simulink model "CurrentControl"  (R2026b)
settings: Solver=VariableStepAuto
undefined symbols (not defined in the file or in its folder): currentCfg, inverterCfg
settings Model: Creator=24322  LastModifiedBy=24322

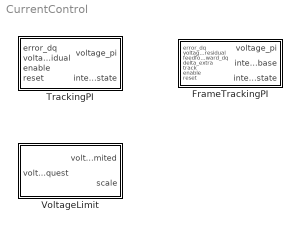
== system CurrentControl ==
  FrameTrackingPI : Subsystem  mask{currentCfg=currentCfg}
      mask prompts: currentCfg "Current controller configuration"
  TrackingPI : Subsystem
  VoltageLimit : Subsystem

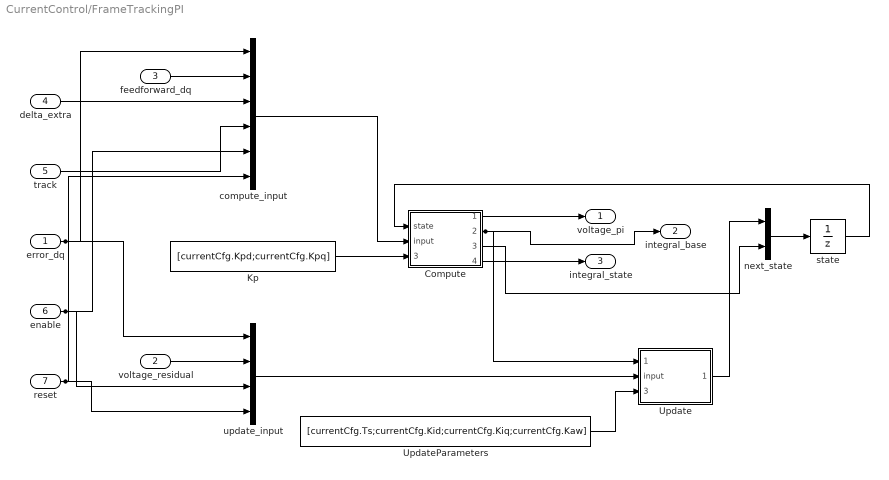
== system CurrentControl/FrameTrackingPI ==
  error_dq : Inport  SampleTime=currentCfg.Ts
  voltage_residual : Inport  Port=2  SampleTime=currentCfg.Ts
  feedforward_dq : Inport  Port=3  SampleTime=currentCfg.Ts
  delta_extra : Inport  Port=4  SampleTime=currentCfg.Ts
  track : Inport  Port=5  SampleTime=currentCfg.Ts
  enable : Inport  Port=6  SampleTime=currentCfg.Ts
  reset : Inport  Port=7  SampleTime=currentCfg.Ts
  Compute : MATLAB Function  TreatAsAtomicUnit=on
  Kp : Constant  Value=[currentCfg.Kpd;currentCfg.Kpq]
  Update : MATLAB Function  TreatAsAtomicUnit=on
  UpdateParameters : Constant  Value=[currentCfg.Ts;currentCfg.Kid;currentCfg.Kiq;currentCfg.Kaw]
  compute_input : Mux  Inputs=6
  next_state : Mux  Inputs=2
  state : UnitDelay  InitialCondition=zeros(8,1)  SampleTime=currentCfg.Ts
  update_input : Mux
  voltage_pi : Outport
  integral_base : Outport  Port=2
  integral_state : Outport  Port=3
  wires:
  voltage_residual/1 -> update_input/2
  reset/1 -> update_input/4, compute_input/6
  enable/1 -> compute_input/5, update_input/3
  track/1 -> compute_input/4
  delta_extra/1 -> compute_input/3
  feedforward_dq/1 -> compute_input/2
  error_dq/1 -> compute_input/1, update_input/1
  Compute/4(integralState) -> integral_state/1
  Compute/1(voltage) -> voltage_pi/1
  next_state/1 -> state/1
  Compute/3(history) -> next_state/2
  Update/1(nextIntegral) -> next_state/1
  UpdateParameters/1 -> Update/3(parameter)
  update_input/1 -> Update/2(input)
  Compute/2(integralBase) -> Update/1(integralBase), integral_base/1
  Kp/1 -> Compute/3(parameter)
  compute_input/1 -> Compute/2(input)
  state/1 -> Compute/1(state)

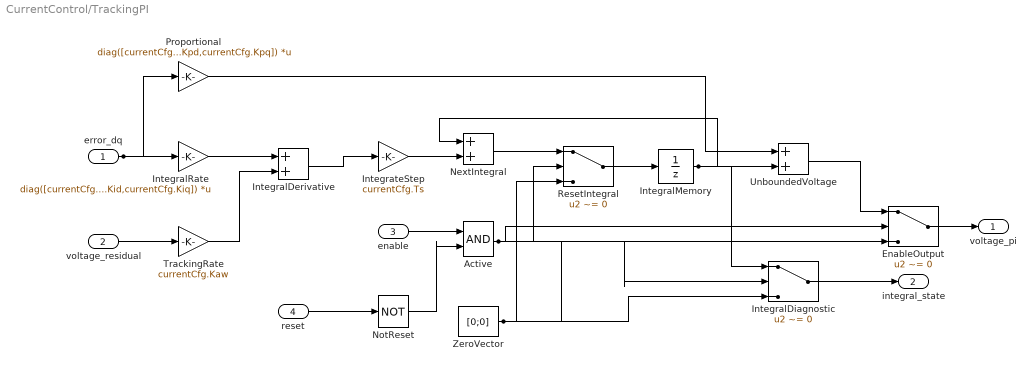
== system CurrentControl/TrackingPI ==
  error_dq : Inport
  voltage_residual : Inport  Port=2
  enable : Inport  Port=3
  reset : Inport  Port=4
  Active : Logic  IconShape=distinctive  AllPortsSameDT=off  OutDataTypeStr=boolean
  EnableOutput : Switch  Criteria=u2 ~= 0  SaturateOnIntegerOverflow=off  InputSameDT=off
  IntegralDerivative : Sum
  IntegralDiagnostic : Switch  Criteria=u2 ~= 0  SaturateOnIntegerOverflow=off  InputSameDT=off
  IntegralMemory : UnitDelay  InitialCondition=[0;0]  SampleTime=currentCfg.Ts
  IntegralRate : Gain  Gain=diag([currentCfg.Kid,currentCfg.Kiq])  Multiplication=Matrix(K*u)
  IntegrateStep : Gain  Gain=currentCfg.Ts
  NextIntegral : Sum
  NotReset : Logic  Operator=NOT  IconShape=distinctive  AllPortsSameDT=off  OutDataTypeStr=boolean
  Proportional : Gain  Gain=diag([currentCfg.Kpd,currentCfg.Kpq])  Multiplication=Matrix(K*u)
  ResetIntegral : Switch  Criteria=u2 ~= 0  SaturateOnIntegerOverflow=off  InputSameDT=off
  TrackingRate : Gain  Gain=currentCfg.Kaw
  UnboundedVoltage : Sum
  ZeroVector : Constant  Value=[0;0]
  voltage_pi : Outport
  integral_state : Outport  Port=2
  wires:
  IntegralDiagnostic/1 -> integral_state/1
  EnableOutput/1 -> voltage_pi/1
  UnboundedVoltage/1 -> EnableOutput/1
  ResetIntegral/1 -> IntegralMemory/1
  ZeroVector/1 -> ResetIntegral/3, EnableOutput/3, IntegralDiagnostic/3
  Active/1 -> ResetIntegral/2, EnableOutput/2, IntegralDiagnostic/2
  NextIntegral/1 -> ResetIntegral/1
  NotReset/1 -> Active/2
  enable/1 -> Active/1
  reset/1 -> NotReset/1
  Proportional/1 -> UnboundedVoltage/1
  IntegrateStep/1 -> NextIntegral/2
  IntegralMemory/1 -> IntegralDiagnostic/1, NextIntegral/1, UnboundedVoltage/2
  IntegralDerivative/1 -> IntegrateStep/1
  TrackingRate/1 -> IntegralDerivative/2
  IntegralRate/1 -> IntegralDerivative/1
  voltage_residual/1 -> TrackingRate/1
  error_dq/1 -> Proportional/1, IntegralRate/1

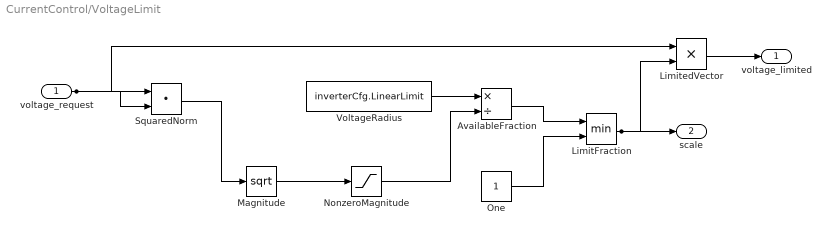
== system CurrentControl/VoltageLimit ==
  voltage_request : Inport
  AvailableFraction : Product  Inputs=*/
  LimitFraction : MinMax  Inputs=2
  LimitedVector : Product
  Magnitude : Math  Operator=sqrt
  NonzeroMagnitude : Saturate  UpperLimit=inf  LowerLimit=1e-12
  One : Constant
  SquaredNorm : DotProduct  OutDataTypeStr=Inherit: Inherit via internal rule
  VoltageRadius : Constant  Value=inverterCfg.LinearLimit
  voltage_limited : Outport
  scale : Outport  Port=2
  wires:
  LimitedVector/1 -> voltage_limited/1
  LimitFraction/1 -> LimitedVector/2, scale/1
  One/1 -> LimitFraction/2
  AvailableFraction/1 -> LimitFraction/1
  NonzeroMagnitude/1 -> AvailableFraction/2
  VoltageRadius/1 -> AvailableFraction/1
  Magnitude/1 -> NonzeroMagnitude/1
  SquaredNorm/1 -> Magnitude/1
  voltage_request/1 -> LimitedVector/1, SquaredNorm/1, SquaredNorm/2

== matlab function CurrentControl/FrameTrackingPI/Update ==
  data: integralBase input; nextIntegral output; input input; parameter input
function nextIntegral=frame_pi_update(integralBase,input,parameter)
%#codegen
%FRAME_PI_UPDATE Residual affects only next Unit Delay state, not present voltage.
% input=[error(2);finalVoltageResidual(2);enable;reset]
% parameter=[Ts;Kid;Kiq;Kaw]
u=cast(input,'like',integralBase);p=cast(parameter,'like',integralBase);
nextIntegral=zeros(2,1,'like',integralBase);
if u(5)<0.5 || u(6)>0.5,return,end
error=[u(1);u(2)];residual=[u(3);u(4)];
nextIntegral=integralBase+p(1)*([p(2);p(3)].*error+p(4)*residual);
end

== matlab function CurrentControl/FrameTrackingPI/Compute ==
  data: state input; voltage output; input input; parameter input; integralBase output; history output; integralState output
function [voltage,integralBase,history,integralState]=frame_pi_compute(state,input,parameter)
%#codegen
%FRAME_PI_COMPUTE Retain physical-error P response while transferring coordinates.
% state=[Iprev(2);Eprev(2);Pprev(2);FFprev(2)]
% input=[error(2);FFnow(2);deltaExtra;track;enable;reset], parameter=[Kpd;Kpq]
u=cast(input,'like',state);p=cast(parameter,'like',state);
voltage=zeros(2,1,'like',state);integralBase=voltage;integralState=voltage;
history=zeros(6,1,'like',state);
if u(7)<0.5 || u(8)>0.5,return,end
error=[u(1);u(2)];feedforward=[u(3);u(4)];
proportional=p.*error;integralState=[state(1);state(2)];
integralBase=integralState;
if u(6)>0.5
    cosine=cos(u(5));sine=sin(u(5));rotation=[cosine,sine;-sine,cosine];
    previousError=[state(3);state(4)];previousP=[state(5);state(6)];
    previousFF=[state(7);state(8)];
    coordinateOnlyP=p.*(rotation*previousError);
    integralBase=rotation*(integralState+previousP+previousFF)-coordinateOnlyP-feedforward;
end
voltage=integralBase+proportional;history=[error;proportional;feedforward];
end
